simulink model "CLSfixed"  (R2023b)
settings: Solver=ode1  StartTime=0.0  StopTime=8000  FixedStep=0.5  RelTol=1e-3
libraries: Libs x311
(part 2 of 2)

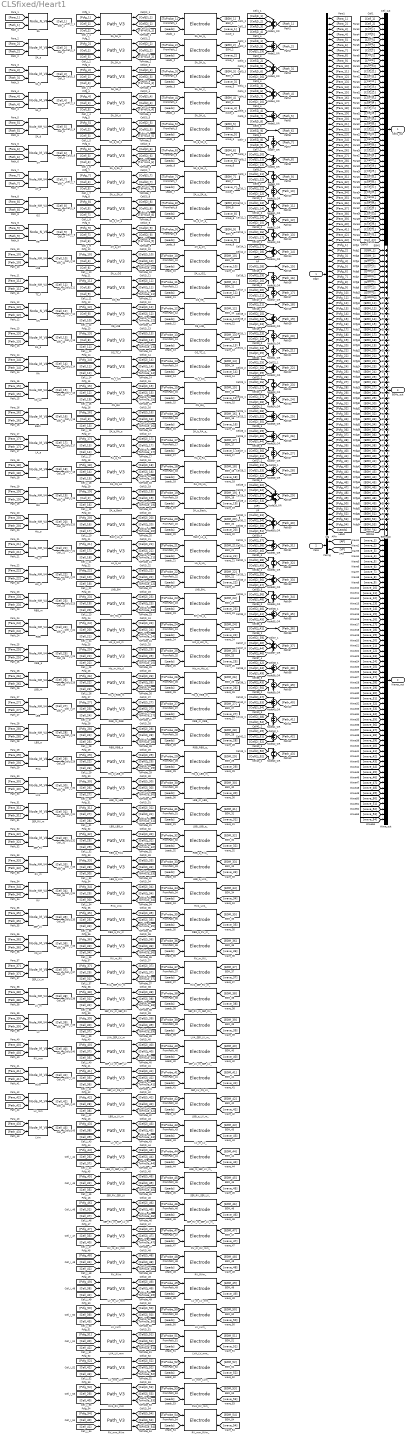
== system CLSfixed/Heart1 ==
  Cfgin : Inport
  Pace : Inport  Port=2
  BH : Libs/Node_NM_V4
  BH_His_p : Libs/Path_V3
  BH_His_p_ : Libs/Electrode
  Bach : Libs/Node_M_V4
  Bach_LA_a : Libs/Path_V3
  Bach_LA_a_ : Libs/Electrode
  CN : Libs/Node_N_V6
  CN_BH : Libs/Path_V3
  CN_BH_ : Libs/Electrode
  CS_LA : Libs/Node_NM_V4
  CS_LV : Libs/Node_M_V4
  CT : Libs/Node_M_V4
  CT_a : Libs/Node_NM_V4
  CT_a_CT : Libs/Path_V3
  CT_a_CT_ : Libs/Electrode
  Cell_out : Mux  Inputs=43
  Cfg : Demux  Outputs=[23,25,25,25,50,25,50,50,23,50,50,23,25,25,50,25,25,25,50,50,50,50,50,50,50,50,50,50,25,25,25,25,50,50,25,25,25,50,50,25,25,25,25,11,11,11,11,11,11,11,11,11,11,11,11,11,11,11,11,11,11,11,11,11,11,11,11,11,11,11,11,11,11,11,11,11,11,11,11,11,11,11,11,11,11,11,11,11,11,11,11,11,11,11,11,11,11,28]
  EGM_out : Sum  Inputs=54
  His_d : Libs/Node_NM_V4
  His_d_LBB_m : Libs/Path_V3
  His_d_LBB_m_ : Libs/Electrode
  His_d_RBB_m : Libs/Path_V3
  His_d_RBB_m_ : Libs/Electrode
  His_m : Libs/Node_NM_V4
  His_m_His_d : Libs/Path_V3
  His_m_His_d_ : Libs/Electrode
  His_p : Libs/Node_NM_V4
  His_p_His_m : Libs/Path_V3
  His_p_His_m_ : Libs/Electrode
  LA : Libs/Node_M_V4
  LA_a : Libs/Node_M_V4
  LA_a_LA : Libs/Path_V3
  LA_a_LA_ : Libs/Electrode
  LBB : Libs/Node_NM_V4
  LBB_LBB_a : Libs/Path_V3
  LBB_LBB_a_ : Libs/Electrode
  LBB_a : Libs/Node_NM_V4
  LBB_a_LVA : Libs/Path_V3
  LBB_a_LVA_ : Libs/Electrode
  LBB_a_LV_m : Libs/Path_V3
  LBB_a_LV_m_ : Libs/Electrode
  LBB_m : Libs/Node_NM_V4
  LBB_m_LBB : Libs/Path_V3
  LBB_m_LBB_ : Libs/Electrode
  LBB_m_SEP_LV_m : Libs/Path_V3
  LBB_m_SEP_LV_m_ : Libs/Electrode
  LNB : Libs/Node_NM_V4
  LNB_BH : Libs/Path_V3
  LNB_BH_ : Libs/Electrode
  LV : Libs/Node_NM_V4
  LVA : Libs/Node_M_V4
  LVA_LV_mm : Libs/Path_V3
  LVA_LV_mm_ : Libs/Electrode
  LVA_SEP_LV_m : Libs/Path_V3
  LVA_SEP_LV_m_ : Libs/Electrode
  LV_LVm : Libs/Path_V3
  LV_LVm_ : Libs/Electrode
  LV_m : Libs/Node_NM_V4
  LV_m_LV : Libs/Path_V3
  LV_m_LV_ : Libs/Electrode
  LV_m_LV_mm : Libs/Path_V3
  LV_m_LV_mm_ : Libs/Electrode
  LV_mm : Libs/Node_M_V4
  LV_mm_LVm : Libs/Path_V3
  LV_mm_LVm_ : Libs/Electrode
  LVm : Libs/Node_M_V4
  Node10_OR : Sum  Inputs=2
  Node11_OR : Sum  Inputs=2
  Node12_OR : Sum  Inputs=2
  Node13_OR : Sum  Inputs=2
  Node14_OR : Sum  Inputs=3
  Node16_OR : Sum  Inputs=2
  Node17_OR : Sum  Inputs=2
  Node19_OR : Sum  Inputs=3
  Node1_OR : Sum  Inputs=4
  Node20_OR : Sum  Inputs=2
  Node21_OR : Sum  Inputs=2
  Node22_OR : Sum  Inputs=3
  Node23_OR : Sum  Inputs=2
  Node24_OR : Sum  Inputs=2
  Node25_OR : Sum  Inputs=3
  Node26_OR : Sum  Inputs=3
  Node27_OR : Sum  Inputs=2
  Node28_OR : Sum  Inputs=3
  Node29_OR : Sum  Inputs=5
  Node2_OR : Sum  Inputs=3
  Node30_OR : Sum  Inputs=4
  Node31_OR : Sum  Inputs=3
  Node32_OR : Sum  Inputs=2
  Node33_OR : Sum  Inputs=3
  Node34_OR : Sum  Inputs=2
  Node35_OR : Sum  Inputs=3
  Node37_OR : Sum  Inputs=4
  Node38_OR : Sum  Inputs=3
  Node39_OR : Sum  Inputs=2
  Node3_OR : Sum  Inputs=4
  Node40_OR : Sum  Inputs=3
  Node41_OR : Sum  Inputs=2
  Node42_OR : Sum  Inputs=3
  Node43_OR : Sum  Inputs=2
  Node4_OR : Sum  Inputs=4
  Node5_OR : Sum  Inputs=3
  Node7_OR : Sum  Inputs=2
  Node8_OR : Sum  Inputs=3
  Node9_OR : Sum  Inputs=2
  OS : Libs/Node_NM_V4
  OS_RE : Libs/Path_V3
  OS_RE_ : Libs/Electrode
  OS_TC_f : Libs/Path_V3
  OS_TC_f_ : Libs/Electrode
  Pacing : Demux  Outputs=2
  RA : Libs/Node_M_V4
  RA_CS_LA : Libs/Path_V3
  RA_CS_LA_ : Libs/Electrode
  RA_a : Libs/Node_M_V4
  RA_a_RA : Libs/Path_V3
  RA_a_RA_ : Libs/Electrode
  RBB : Libs/Node_NM_V4
  RBB_RBB_a : Libs/Path_V3
  RBB_RBB_a_ : Libs/Electrode
  RBB_a : Libs/Node_NM_V4
  RBB_a_RVA : Libs/Path_V3
  RBB_a_RVA_ : Libs/Electrode
  RBB_a_RV_m : Libs/Path_V3
  RBB_a_RV_m_ : Libs/Electrode
  RBB_m : Libs/Node_NM_V4
  RBB_m_RBB : Libs/Path_V3
  RBB_m_RBB_ : Libs/Electrode
  RE : Libs/Node_N_V6
  RE_LNB : Libs/Path_V3
  RE_LNB_ : Libs/Electrode
  RV : Libs/Node_NM_V4
  RVA : Libs/Node_M_V4
  RVA_LVA : Libs/Path_V3
  RVA_LVA_ : Libs/Electrode
  RVA_RV_mm : Libs/Path_V3
  RVA_RV_mm_ : Libs/Electrode
  RVA_SEP_RV_m : Libs/Path_V3
  RVA_SEP_RV_m_ : Libs/Electrode
  RV_RVm : Libs/Path_V3
  RV_RVm_ : Libs/Electrode
  RV_m : Libs/Node_NM_V4
  RV_m_RV : Libs/Path_V3
  RV_m_RV_ : Libs/Electrode
  RV_m_RV_mm : Libs/Path_V3
  RV_m_RV_mm_ : Libs/Electrode
  RV_mm : Libs/Node_M_V4
  RV_mm_RVm : Libs/Path_V3
  RV_mm_RVm_ : Libs/Electrode
  RVm : Libs/Node_M_V4
  SA : Libs/Node_N_V6
  SA_SA_a : Libs/Path_V3
  SA_SA_a_ : Libs/Electrode
  SA_SA_b : Libs/Path_V3
  SA_SA_b_ : Libs/Electrode
  SA_SA_c : Libs/Path_V3
  SA_SA_c_ : Libs/Electrode
  SA_SA_d : Libs/Path_V3
  SA_SA_d_ : Libs/Electrode
  SA_a : Libs/Node_M_V4
  SA_a_Bach : Libs/Path_V3
  SA_a_Bach_ : Libs/Electrode
  SA_a_SA_b : Libs/Path_V3
  SA_a_SA_b_ : Libs/Electrode
  SA_b : Libs/Node_M_V4
  SA_b_RA_a : Libs/Path_V3
  SA_b_RA_a_ : Libs/Electrode
  SA_b_SA_c : Libs/Path_V3
  SA_b_SA_c_ : Libs/Electrode
  SA_c : Libs/Node_M_V4
  SA_c_OS : Libs/Path_V3
  SA_c_OS_ : Libs/Electrode
  SA_c_SA_d : Libs/Path_V3
  SA_c_SA_d_ : Libs/Electrode
  SA_d : Libs/Node_NM_V4
  SA_d_CT_a : Libs/Path_V3
  SA_d_CT_a_ : Libs/Electrode
  SEP_LV : Libs/Node_M_V4
  SEP_LV_CS_LV : Libs/Path_V3
  SEP_LV_CS_LV_ : Libs/Electrode
  SEP_LV_m : Libs/Node_M_V4
  SEP_LV_m_SEP_LV : Libs/Path_V3
  SEP_LV_m_SEP_LV_ : Libs/Electrode
  SEP_RV : Libs/Node_M_V4
  SEP_RV_SEP_LV : Libs/Path_V3
  SEP_RV_SEP_LV_ : Libs/Electrode
  SEP_RV_m : Libs/Node_M_V4
  SEP_RV_m_SEP_LV_m : Libs/Path_V3
  SEP_RV_m_SEP_LV_m_ : Libs/Electrode
  SEP_RV_m_SEP_RV : Libs/Path_V3
  SEP_RV_m_SEP_RV_ : Libs/Electrode
  TC_f : Libs/Node_NM_V4
  TC_f_CN : Libs/Path_V3
  TC_f_CN_ : Libs/Electrode
  Wave_out : Mux  Inputs=54
  Cells_out : Outport
  Waves_out : Outport  Port=2
  EGMs_out : Outport  Port=3
  wires:
  SA/1 -> [Cell_1]
  [Para_1] -> SA/1
  [Path_1] -> SA/2
  SA_a/1 -> [Cell_2]
  [Para_2] -> SA_a/1
  [Path_2] -> SA_a/2
  SA_b/1 -> [Cell_3]
  [Para_3] -> SA_b/1
  [Path_3] -> SA_b/2
  SA_c/1 -> [Cell_4]
  [Para_4] -> SA_c/1
  [Path_4] -> SA_c/2
  SA_d/1 -> [Cell_5]
  [Para_5] -> SA_d/1
  [Path_5] -> SA_d/2
  CT/1 -> [Cell_6]
  [Para_6] -> CT/1
  [Path_6] -> CT/2
  CT_a/1 -> [Cell_7]
  [Para_7] -> CT_a/1
  [Path_7] -> CT_a/2
  OS/1 -> [Cell_8]
  [Para_8] -> OS/1
  [Path_8] -> OS/2
  RE/1 -> [Cell_9]
  [Para_9] -> RE/1
  [Path_9] -> RE/2
  LNB/1 -> [Cell_10]
  [Para_10] -> LNB/1
  [Path_10] -> LNB/2
  TC_f/1 -> [Cell_11]
  [Para_11] -> TC_f/1
  [Path_11] -> TC_f/2
  CN/1 -> [Cell_12]
  [Para_12] -> CN/1
  [Path_12] -> CN/2
  RA_a/1 -> [Cell_13]
  [Para_13] -> RA_a/1
  [Path_13] -> RA_a/2
  RA/1 -> [Cell_14]
  [Para_14] -> RA/1
  [Path_14] -> RA/2
  CS_LA/1 -> [Cell_15]
  [Para_15] -> CS_LA/1
  [Path_15] -> CS_LA/2
  Bach/1 -> [Cell_16]
  [Para_16] -> Bach/1
  [Path_16] -> Bach/2
  LA_a/1 -> [Cell_17]
  [Para_17] -> LA_a/1
  [Path_17] -> LA_a/2
  LA/1 -> [Cell_18]
  [Para_18] -> LA/1
  [Path_18] -> LA/2
  BH/1 -> [Cell_19]
  [Para_19] -> BH/1
  [Path_19] -> BH/2
  His_p/1 -> [Cell_20]
  [Para_20] -> His_p/1
  [Path_20] -> His_p/2
  His_m/1 -> [Cell_21]
  [Para_21] -> His_m/1
  [Path_21] -> His_m/2
  His_d/1 -> [Cell_22]
  [Para_22] -> His_d/1
  [Path_22] -> His_d/2
  RBB_m/1 -> [Cell_23]
  [Para_23] -> RBB_m/1
  [Path_23] -> RBB_m/2
  RBB/1 -> [Cell_24]
  [Para_24] -> RBB/1
  [Path_24] -> RBB/2
  RBB_a/1 -> [Cell_25]
  [Para_25] -> RBB_a/1
  [Path_25] -> RBB_a/2
  LBB_m/1 -> [Cell_26]
  [Para_26] -> LBB_m/1
  [Path_26] -> LBB_m/2
  LBB/1 -> [Cell_27]
  [Para_27] -> LBB/1
  [Path_27] -> LBB/2
  LBB_a/1 -> [Cell_28]
  [Para_28] -> LBB_a/1
  [Path_28] -> LBB_a/2
  RVA/1 -> [Cell_29]
  [Para_29] -> RVA/1
  [Path_29] -> RVA/2
  LVA/1 -> [Cell_30]
  [Para_30] -> LVA/1
  [Path_30] -> LVA/2
  SEP_RV_m/1 -> [Cell_31]
  [Para_31] -> SEP_RV_m/1
  [Path_31] -> SEP_RV_m/2
  SEP_RV/1 -> [Cell_32]
  [Para_32] -> SEP_RV/1
  [Path_32] -> SEP_RV/2
  RV_m/1 -> [Cell_33]
  [Para_33] -> RV_m/1
  [Path_33] -> RV_m/2
  RV/1 -> [Cell_34]
  [Para_34] -> RV/1
  [Path_34] -> RV/2
  SEP_LV/1 -> [Cell_35]
  [Para_35] -> SEP_LV/1
  [Path_35] -> SEP_LV/2
  CS_LV/1 -> [Cell_36]
  [Para_36] -> CS_LV/1
  [Path_36] -> CS_LV/2
  SEP_LV_m/1 -> [Cell_37]
  [Para_37] -> SEP_LV_m/1
  [Path_37] -> SEP_LV_m/2
  LV_m/1 -> [Cell_38]
  [Para_38] -> LV_m/1
  [Path_38] -> LV_m/2
  LV/1 -> [Cell_39]
  [Para_39] -> LV/1
  [Path_39] -> LV/2
  RV_mm/1 -> [Cell_40]
  [Para_40] -> RV_mm/1
  [Path_40] -> RV_mm/2
  RVm/1 -> [Cell_41]
  [Para_41] -> RVm/1
  [Path_41] -> RVm/2
  LV_mm/1 -> [Cell_42]
  [Para_42] -> LV_mm/1
  [Path_42] -> LV_mm/2
  LVm/1 -> [Cell_43]
  [Para_43] -> LVm/1
  [Path_43] -> LVm/2
  SA_SA_a/1 -> [Cellj2i_1]
  SA_SA_a/2 -> [Celli2j_1]
  SA_SA_a/3 -> [ToProbe_1]
  [Pcfg_1] -> SA_SA_a/1
  [Cell_1] -> SA_SA_a/2
  [Cell_2] -> SA_SA_a/3
  SA_SA_b/1 -> [Cellj2i_2]
  SA_SA_b/2 -> [Celli2j_2]
  SA_SA_b/3 -> [ToProbe_2]
  [Pcfg_2] -> SA_SA_b/1
  [Cell_1] -> SA_SA_b/2
  [Cell_3] -> SA_SA_b/3
  SA_SA_c/1 -> [Cellj2i_3]
  SA_SA_c/2 -> [Celli2j_3]
  SA_SA_c/3 -> [ToProbe_3]
  [Pcfg_3] -> SA_SA_c/1
  [Cell_1] -> SA_SA_c/2
  [Cell_4] -> SA_SA_c/3
  SA_SA_d/1 -> [Cellj2i_4]
  SA_SA_d/2 -> [Celli2j_4]
  SA_SA_d/3 -> [ToProbe_4]
  [Pcfg_4] -> SA_SA_d/1
  [Cell_1] -> SA_SA_d/2
  [Cell_5] -> SA_SA_d/3
  SA_a_SA_b/1 -> [Cellj2i_5]
  SA_a_SA_b/2 -> [Celli2j_5]
  SA_a_SA_b/3 -> [ToProbe_5]
  [Pcfg_5] -> SA_a_SA_b/1
  [Cell_2] -> SA_a_SA_b/2
  [Cell_3] -> SA_a_SA_b/3
  SA_b_SA_c/1 -> [Cellj2i_6]
  SA_b_SA_c/2 -> [Celli2j_6]
  SA_b_SA_c/3 -> [ToProbe_6]
  [Pcfg_6] -> SA_b_SA_c/1
  [Cell_3] -> SA_b_SA_c/2
  [Cell_4] -> SA_b_SA_c/3
  SA_c_SA_d/1 -> [Cellj2i_7]
  SA_c_SA_d/2 -> [Celli2j_7]
  SA_c_SA_d/3 -> [ToProbe_7]
  [Pcfg_7] -> SA_c_SA_d/1
  [Cell_4] -> SA_c_SA_d/2
  [Cell_5] -> SA_c_SA_d/3
  SA_d_CT_a/1 -> [Cellj2i_8]
  SA_d_CT_a/2 -> [Celli2j_8]
  SA_d_CT_a/3 -> [ToProbe_8]
  [Pcfg_8] -> SA_d_CT_a/1
  [Cell_5] -> SA_d_CT_a/2
  [Cell_7] -> SA_d_CT_a/3
  CT_a_CT/1 -> [Cellj2i_9]
  CT_a_CT/2 -> [Celli2j_9]
  CT_a_CT/3 -> [ToProbe_9]
  [Pcfg_9] -> CT_a_CT/1
  [Cell_7] -> CT_a_CT/2
  [Cell_6] -> CT_a_CT/3
  SA_c_OS/1 -> [Cellj2i_10]
  SA_c_OS/2 -> [Celli2j_10]
  SA_c_OS/3 -> [ToProbe_10]
  [Pcfg_10] -> SA_c_OS/1
  [Cell_4] -> SA_c_OS/2
  [Cell_8] -> SA_c_OS/3
  OS_RE/1 -> [Cellj2i_11]
  OS_RE/2 -> [Celli2j_11]
  OS_RE/3 -> [ToProbe_11]
  [Pcfg_11] -> OS_RE/1
  [Cell_8] -> OS_RE/2
  [Cell_9] -> OS_RE/3
  RE_LNB/1 -> [Cellj2i_12]
  RE_LNB/2 -> [Celli2j_12]
  RE_LNB/3 -> [ToProbe_12]
  [Pcfg_12] -> RE_LNB/1
  [Cell_9] -> RE_LNB/2
  [Cell_10] -> RE_LNB/3
  OS_TC_f/1 -> [Cellj2i_13]
  OS_TC_f/2 -> [Celli2j_13]
  OS_TC_f/3 -> [ToProbe_13]
  [Pcfg_13] -> OS_TC_f/1
  [Cell_8] -> OS_TC_f/2
  [Cell_11] -> OS_TC_f/3
  TC_f_CN/1 -> [Cellj2i_14]
  TC_f_CN/2 -> [Celli2j_14]
  TC_f_CN/3 -> [ToProbe_14]
  [Pcfg_14] -> TC_f_CN/1
  [Cell_11] -> TC_f_CN/2
  [Cell_12] -> TC_f_CN/3
  CN_BH/1 -> [Cellj2i_15]
  CN_BH/2 -> [Celli2j_15]
  CN_BH/3 -> [ToProbe_15]
  [Pcfg_15] -> CN_BH/1
  [Cell_12] -> CN_BH/2
  [Cell_19] -> CN_BH/3
  SA_b_RA_a/1 -> [Cellj2i_16]
  SA_b_RA_a/2 -> [Celli2j_16]
  SA_b_RA_a/3 -> [ToProbe_16]
  [Pcfg_16] -> SA_b_RA_a/1
  [Cell_3] -> SA_b_RA_a/2
  [Cell_13] -> SA_b_RA_a/3
  RA_a_RA/1 -> [Cellj2i_17]
  RA_a_RA/2 -> [Celli2j_17]
  RA_a_RA/3 -> [ToProbe_17]
  [Pcfg_17] -> RA_a_RA/1
  [Cell_13] -> RA_a_RA/2
  [Cell_14] -> RA_a_RA/3
  RA_CS_LA/1 -> [Cellj2i_18]
  RA_CS_LA/2 -> [Celli2j_18]
  RA_CS_LA/3 -> [ToProbe_18]
  [Pcfg_18] -> RA_CS_LA/1
  [Cell_14] -> RA_CS_LA/2
  [Cell_15] -> RA_CS_LA/3
  SA_a_Bach/1 -> [Cellj2i_19]
  SA_a_Bach/2 -> [Celli2j_19]
  SA_a_Bach/3 -> [ToProbe_19]
  [Pcfg_19] -> SA_a_Bach/1
  [Cell_2] -> SA_a_Bach/2
  [Cell_16] -> SA_a_Bach/3
  Bach_LA_a/1 -> [Cellj2i_20]
  Bach_LA_a/2 -> [Celli2j_20]
  Bach_LA_a/3 -> [ToProbe_20]
  [Pcfg_20] -> Bach_LA_a/1
  [Cell_16] -> Bach_LA_a/2
  [Cell_17] -> Bach_LA_a/3
  LA_a_LA/1 -> [Cellj2i_21]
  LA_a_LA/2 -> [Celli2j_21]
  LA_a_LA/3 -> [ToProbe_21]
  [Pcfg_21] -> LA_a_LA/1
  [Cell_17] -> LA_a_LA/2
  [Cell_18] -> LA_a_LA/3
  LNB_BH/1 -> [Cellj2i_22]
  LNB_BH/2 -> [Celli2j_22]
  LNB_BH/3 -> [ToProbe_22]
  [Pcfg_22] -> LNB_BH/1
  [Cell_10] -> LNB_BH/2
  [Cell_19] -> LNB_BH/3
  BH_His_p/1 -> [Cellj2i_23]
  BH_His_p/2 -> [Celli2j_23]
  BH_His_p/3 -> [ToProbe_23]
  [Pcfg_23] -> BH_His_p/1
  [Cell_19] -> BH_His_p/2
  [Cell_20] -> BH_His_p/3
  His_p_His_m/1 -> [Cellj2i_24]
  His_p_His_m/2 -> [Celli2j_24]
  His_p_His_m/3 -> [ToProbe_24]
  [Pcfg_24] -> His_p_His_m/1
  [Cell_20] -> His_p_His_m/2
  [Cell_21] -> His_p_His_m/3
  His_m_His_d/1 -> [Cellj2i_25]
  His_m_His_d/2 -> [Celli2j_25]
  His_m_His_d/3 -> [ToProbe_25]
  [Pcfg_25] -> His_m_His_d/1
  [Cell_21] -> His_m_His_d/2
  [Cell_22] -> His_m_His_d/3
  His_d_RBB_m/1 -> [Cellj2i_26]
  His_d_RBB_m/2 -> [Celli2j_26]
  His_d_RBB_m/3 -> [ToProbe_26]
  [Pcfg_26] -> His_d_RBB_m/1
  [Cell_22] -> His_d_RBB_m/2
  [Cell_23] -> His_d_RBB_m/3
  RBB_m_RBB/1 -> [Cellj2i_27]
  RBB_m_RBB/2 -> [Celli2j_27]
  RBB_m_RBB/3 -> [ToProbe_27]
  [Pcfg_27] -> RBB_m_RBB/1
  [Cell_23] -> RBB_m_RBB/2
  [Cell_24] -> RBB_m_RBB/3
  RBB_RBB_a/1 -> [Cellj2i_28]
  RBB_RBB_a/2 -> [Celli2j_28]
  RBB_RBB_a/3 -> [ToProbe_28]
  [Pcfg_28] -> RBB_RBB_a/1
  [Cell_24] -> RBB_RBB_a/2
  [Cell_25] -> RBB_RBB_a/3
  His_d_LBB_m/1 -> [Cellj2i_29]
  His_d_LBB_m/2 -> [Celli2j_29]
  His_d_LBB_m/3 -> [ToProbe_29]
  [Pcfg_29] -> His_d_LBB_m/1
  [Cell_22] -> His_d_LBB_m/2
  [Cell_26] -> His_d_LBB_m/3
  LBB_m_LBB/1 -> [Cellj2i_30]
  LBB_m_LBB/2 -> [Celli2j_30]
  LBB_m_LBB/3 -> [ToProbe_30]
  [Pcfg_30] -> LBB_m_LBB/1
  [Cell_26] -> LBB_m_LBB/2
  [Cell_27] -> LBB_m_LBB/3
  LBB_LBB_a/1 -> [Cellj2i_31]
  LBB_LBB_a/2 -> [Celli2j_31]
  LBB_LBB_a/3 -> [ToProbe_31]
  [Pcfg_31] -> LBB_LBB_a/1
  [Cell_27] -> LBB_LBB_a/2
  [Cell_28] -> LBB_LBB_a/3
  RBB_a_RVA/1 -> [Cellj2i_32]
  RBB_a_RVA/2 -> [Celli2j_32]
  RBB_a_RVA/3 -> [ToProbe_32]
  [Pcfg_32] -> RBB_a_RVA/1
  [Cell_25] -> RBB_a_RVA/2
  [Cell_29] -> RBB_a_RVA/3
  LBB_a_LVA/1 -> [Cellj2i_33]
  LBB_a_LVA/2 -> [Celli2j_33]
  LBB_a_LVA/3 -> [ToProbe_33]
  [Pcfg_33] -> LBB_a_LVA/1
  [Cell_28] -> LBB_a_LVA/2
  [Cell_30] -> LBB_a_LVA/3
  RVA_LVA/1 -> [Cellj2i_34]
  RVA_LVA/2 -> [Celli2j_34]
  RVA_LVA/3 -> [ToProbe_34]
  [Pcfg_34] -> RVA_LVA/1
  [Cell_29] -> RVA_LVA/2
  [Cell_30] -> RVA_LVA/3
  RBB_a_RV_m/1 -> [Cellj2i_35]
  RBB_a_RV_m/2 -> [Celli2j_35]
  RBB_a_RV_m/3 -> [ToProbe_35]
  [Pcfg_35] -> RBB_a_RV_m/1
  [Cell_25] -> RBB_a_RV_m/2
  [Cell_33] -> RBB_a_RV_m/3
  RV_m_RV/1 -> [Cellj2i_36]
  RV_m_RV/2 -> [Celli2j_36]
  RV_m_RV/3 -> [ToProbe_36]
  [Pcfg_36] -> RV_m_RV/1
  [Cell_33] -> RV_m_RV/2
  [Cell_34] -> RV_m_RV/3
  RVA_SEP_RV_m/1 -> [Cellj2i_37]
  RVA_SEP_RV_m/2 -> [Celli2j_37]
  RVA_SEP_RV_m/3 -> [ToProbe_37]
  [Pcfg_37] -> RVA_SEP_RV_m/1
  [Cell_29] -> RVA_SEP_RV_m/2
  [Cell_31] -> RVA_SEP_RV_m/3
  SEP_RV_m_SEP_RV/1 -> [Cellj2i_38]
  SEP_RV_m_SEP_RV/2 -> [Celli2j_38]
  SEP_RV_m_SEP_RV/3 -> [ToProbe_38]
  [Pcfg_38] -> SEP_RV_m_SEP_RV/1
  [Cell_31] -> SEP_RV_m_SEP_RV/2
  [Cell_32] -> SEP_RV_m_SEP_RV/3
  LVA_SEP_LV_m/1 -> [Cellj2i_39]
  LVA_SEP_LV_m/2 -> [Celli2j_39]
  LVA_SEP_LV_m/3 -> [ToProbe_39]
  [Pcfg_39] -> LVA_SEP_LV_m/1
  [Cell_30] -> LVA_SEP_LV_m/2
  [Cell_37] -> LVA_SEP_LV_m/3
  SEP_LV_m_SEP_LV/1 -> [Cellj2i_40]
  SEP_LV_m_SEP_LV/2 -> [Celli2j_40]
  SEP_LV_m_SEP_LV/3 -> [ToProbe_40]
  [Pcfg_40] -> SEP_LV_m_SEP_LV/1
  [Cell_37] -> SEP_LV_m_SEP_LV/2
  [Cell_35] -> SEP_LV_m_SEP_LV/3
  SEP_LV_CS_LV/1 -> [Cellj2i_41]
  SEP_LV_CS_LV/2 -> [Celli2j_41]
  SEP_LV_CS_LV/3 -> [ToProbe_41]
  [Pcfg_41] -> SEP_LV_CS_LV/1
  [Cell_35] -> SEP_LV_CS_LV/2
  [Cell_36] -> SEP_LV_CS_LV/3
  LBB_a_LV_m/1 -> [Cellj2i_42]
  LBB_a_LV_m/2 -> [Celli2j_42]
  LBB_a_LV_m/3 -> [ToProbe_42]
  [Pcfg_42] -> LBB_a_LV_m/1
  [Cell_28] -> LBB_a_LV_m/2
  [Cell_38] -> LBB_a_LV_m/3
  LV_m_LV/1 -> [Cellj2i_43]
  LV_m_LV/2 -> [Celli2j_43]
  LV_m_LV/3 -> [ToProbe_43]
  [Pcfg_43] -> LV_m_LV/1
  [Cell_38] -> LV_m_LV/2
  [Cell_39] -> LV_m_LV/3
  LBB_m_SEP_LV_m/1 -> [Cellj2i_44]
  LBB_m_SEP_LV_m/2 -> [Celli2j_44]
  LBB_m_SEP_LV_m/3 -> [ToProbe_44]
  [Pcfg_44] -> LBB_m_SEP_LV_m/1
  [Cell_26] -> LBB_m_SEP_LV_m/2
  [Cell_37] -> LBB_m_SEP_LV_m/3
  SEP_RV_SEP_LV/1 -> [Cellj2i_45]
  SEP_RV_SEP_LV/2 -> [Celli2j_45]
  SEP_RV_SEP_LV/3 -> [ToProbe_45]
  [Pcfg_45] -> SEP_RV_SEP_LV/1
  [Cell_32] -> SEP_RV_SEP_LV/2
  [Cell_35] -> SEP_RV_SEP_LV/3
  SEP_RV_m_SEP_LV_m/1 -> [Cellj2i_46]
  SEP_RV_m_SEP_LV_m/2 -> [Celli2j_46]
  SEP_RV_m_SEP_LV_m/3 -> [ToProbe_46]
  [Pcfg_46] -> SEP_RV_m_SEP_LV_m/1
  [Cell_31] -> SEP_RV_m_SEP_LV_m/2
  [Cell_37] -> SEP_RV_m_SEP_LV_m/3
  RV_m_RV_mm/1 -> [Cellj2i_47]
  RV_m_RV_mm/2 -> [Celli2j_47]
  RV_m_RV_mm/3 -> [ToProbe_47]
  [Pcfg_47] -> RV_m_RV_mm/1
  [Cell_33] -> RV_m_RV_mm/2
  [Cell_40] -> RV_m_RV_mm/3
  RV_RVm/1 -> [Cellj2i_48]
  RV_RVm/2 -> [Celli2j_48]
  RV_RVm/3 -> [ToProbe_48]
  [Pcfg_48] -> RV_RVm/1
  [Cell_34] -> RV_RVm/2
  [Cell_41] -> RV_RVm/3
  LV_m_LV_mm/1 -> [Cellj2i_49]
  LV_m_LV_mm/2 -> [Celli2j_49]
  LV_m_LV_mm/3 -> [ToProbe_49]
  [Pcfg_49] -> LV_m_LV_mm/1
  [Cell_38] -> LV_m_LV_mm/2
  [Cell_42] -> LV_m_LV_mm/3
  LV_LVm/1 -> [Cellj2i_50]
  LV_LVm/2 -> [Celli2j_50]
  LV_LVm/3 -> [ToProbe_50]
  [Pcfg_50] -> LV_LVm/1
  [Cell_39] -> LV_LVm/2
  [Cell_43] -> LV_LVm/3
  LVA_LV_mm/1 -> [Cellj2i_51]
  LVA_LV_mm/2 -> [Celli2j_51]
  LVA_LV_mm/3 -> [ToProbe_51]
  [Pcfg_51] -> LVA_LV_mm/1
  [Cell_30] -> LVA_LV_mm/2
  [Cell_42] -> LVA_LV_mm/3
  LV_mm_LVm/1 -> [Cellj2i_52]
  LV_mm_LVm/2 -> [Celli2j_52]
  LV_mm_LVm/3 -> [ToProbe_52]
  [Pcfg_52] -> LV_mm_LVm/1
  [Cell_42] -> LV_mm_LVm/2
  [Cell_43] -> LV_mm_LVm/3
  RVA_RV_mm/1 -> [Cellj2i_53]
  RVA_RV_mm/2 -> [Celli2j_53]
  RVA_RV_mm/3 -> [ToProbe_53]
  [Pcfg_53] -> RVA_RV_mm/1
  [Cell_29] -> RVA_RV_mm/2
  [Cell_40] -> RVA_RV_mm/3
  RV_mm_RVm/1 -> [Cellj2i_54]
  RV_mm_RVm/2 -> [Celli2j_54]
  RV_mm_RVm/3 -> [ToProbe_54]
  [Pcfg_54] -> RV_mm_RVm/1
  [Cell_40] -> RV_mm_RVm/2
  [Cell_41] -> RV_mm_RVm/3
  SA_SA_a_/1 -> [EGM_1]
  SA_SA_a_/2 -> [wave_1]
  [ToProbe_1] -> SA_SA_a_/1
  [Leads] -> SA_SA_a_/2
  SA_SA_b_/1 -> [EGM_2]
  SA_SA_b_/2 -> [wave_2]
  [ToProbe_2] -> SA_SA_b_/1
  [Leads] -> SA_SA_b_/2
  SA_SA_c_/1 -> [EGM_3]
  SA_SA_c_/2 -> [wave_3]
  [ToProbe_3] -> SA_SA_c_/1
  [Leads] -> SA_SA_c_/2
  SA_SA_d_/1 -> [EGM_4]
  SA_SA_d_/2 -> [wave_4]
  [ToProbe_4] -> SA_SA_d_/1
  [Leads] -> SA_SA_d_/2
  SA_a_SA_b_/1 -> [EGM_5]
  SA_a_SA_b_/2 -> [wave_5]
  [ToProbe_5] -> SA_a_SA_b_/1
  [Leads] -> SA_a_SA_b_/2
  SA_b_SA_c_/1 -> [EGM_6]
  SA_b_SA_c_/2 -> [wave_6]
  [ToProbe_6] -> SA_b_SA_c_/1
  [Leads] -> SA_b_SA_c_/2
  SA_c_SA_d_/1 -> [EGM_7]
  SA_c_SA_d_/2 -> [wave_7]
  [ToProbe_7] -> SA_c_SA_d_/1
  [Leads] -> SA_c_SA_d_/2
  SA_d_CT_a_/1 -> [EGM_8]
  SA_d_CT_a_/2 -> [wave_8]
  [ToProbe_8] -> SA_d_CT_a_/1
  [Leads] -> SA_d_CT_a_/2
  CT_a_CT_/1 -> [EGM_9]
  CT_a_CT_/2 -> [wave_9]
  [ToProbe_9] -> CT_a_CT_/1
  [Leads] -> CT_a_CT_/2
  SA_c_OS_/1 -> [EGM_10]
  SA_c_OS_/2 -> [wave_10]
  [ToProbe_10] -> SA_c_OS_/1
  [Leads] -> SA_c_OS_/2
  OS_RE_/1 -> [EGM_11]
  OS_RE_/2 -> [wave_11]
  [ToProbe_11] -> OS_RE_/1
  [Leads] -> OS_RE_/2
  RE_LNB_/1 -> [EGM_12]
  RE_LNB_/2 -> [wave_12]
  [ToProbe_12] -> RE_LNB_/1
  [Leads] -> RE_LNB_/2
  OS_TC_f_/1 -> [EGM_13]
  OS_TC_f_/2 -> [wave_13]
  [ToProbe_13] -> OS_TC_f_/1
  [Leads] -> OS_TC_f_/2
  TC_f_CN_/1 -> [EGM_14]
  TC_f_CN_/2 -> [wave_14]
  [ToProbe_14] -> TC_f_CN_/1
  [Leads] -> TC_f_CN_/2
  CN_BH_/1 -> [EGM_15]
  CN_BH_/2 -> [wave_15]
  [ToProbe_15] -> CN_BH_/1
  [Leads] -> CN_BH_/2
  SA_b_RA_a_/1 -> [EGM_16]
  SA_b_RA_a_/2 -> [wave_16]
  [ToProbe_16] -> SA_b_RA_a_/1
  [Leads] -> SA_b_RA_a_/2
  RA_a_RA_/1 -> [EGM_17]
  RA_a_RA_/2 -> [wave_17]
  [ToProbe_17] -> RA_a_RA_/1
  [Leads] -> RA_a_RA_/2
  RA_CS_LA_/1 -> [EGM_18]
  RA_CS_LA_/2 -> [wave_18]
  [ToProbe_18] -> RA_CS_LA_/1
  [Leads] -> RA_CS_LA_/2
  SA_a_Bach_/1 -> [EGM_19]
  SA_a_Bach_/2 -> [wave_19]
  [ToProbe_19] -> SA_a_Bach_/1
  [Leads] -> SA_a_Bach_/2
  Bach_LA_a_/1 -> [EGM_20]
  Bach_LA_a_/2 -> [wave_20]
  [ToProbe_20] -> Bach_LA_a_/1
  [Leads] -> Bach_LA_a_/2
  LA_a_LA_/1 -> [EGM_21]
  LA_a_LA_/2 -> [wave_21]
  [ToProbe_21] -> LA_a_LA_/1
  [Leads] -> LA_a_LA_/2
  LNB_BH_/1 -> [EGM_22]
  LNB_BH_/2 -> [wave_22]
  [ToProbe_22] -> LNB_BH_/1
  [Leads] -> LNB_BH_/2
  BH_His_p_/1 -> [EGM_23]
  BH_His_p_/2 -> [wave_23]
  [ToProbe_23] -> BH_His_p_/1
  [Leads] -> BH_His_p_/2
  His_p_His_m_/1 -> [EGM_24]
  His_p_His_m_/2 -> [wave_24]
  [ToProbe_24] -> His_p_His_m_/1
  [Leads] -> His_p_His_m_/2
  His_m_His_d_/1 -> [EGM_25]
  His_m_His_d_/2 -> [wave_25]
  [ToProbe_25] -> His_m_His_d_/1
  [Leads] -> His_m_His_d_/2
  His_d_RBB_m_/1 -> [EGM_26]
  His_d_RBB_m_/2 -> [wave_26]
  [ToProbe_26] -> His_d_RBB_m_/1
  [Leads] -> His_d_RBB_m_/2
  RBB_m_RBB_/1 -> [EGM_27]
  RBB_m_RBB_/2 -> [wave_27]
  [ToProbe_27] -> RBB_m_RBB_/1
  [Leads] -> RBB_m_RBB_/2
  RBB_RBB_a_/1 -> [EGM_28]
  RBB_RBB_a_/2 -> [wave_28]
  [ToProbe_28] -> RBB_RBB_a_/1
  [Leads] -> RBB_RBB_a_/2
  His_d_LBB_m_/1 -> [EGM_29]
  His_d_LBB_m_/2 -> [wave_29]
  [ToProbe_29] -> His_d_LBB_m_/1
  [Leads] -> His_d_LBB_m_/2
  LBB_m_LBB_/1 -> [EGM_30]
  LBB_m_LBB_/2 -> [wave_30]
  [ToProbe_30] -> LBB_m_LBB_/1
  [Leads] -> LBB_m_LBB_/2
  LBB_LBB_a_/1 -> [EGM_31]
  LBB_LBB_a_/2 -> [wave_31]
  [ToProbe_31] -> LBB_LBB_a_/1
  [Leads] -> LBB_LBB_a_/2
  RBB_a_RVA_/1 -> [EGM_32]
  RBB_a_RVA_/2 -> [wave_32]
  [ToProbe_32] -> RBB_a_RVA_/1
  [Leads] -> RBB_a_RVA_/2
  LBB_a_LVA_/1 -> [EGM_33]
  LBB_a_LVA_/2 -> [wave_33]
  [ToProbe_33] -> LBB_a_LVA_/1
  [Leads] -> LBB_a_LVA_/2
  RVA_LVA_/1 -> [EGM_34]
  RVA_LVA_/2 -> [wave_34]
  [ToProbe_34] -> RVA_LVA_/1
  [Leads] -> RVA_LVA_/2
  RBB_a_RV_m_/1 -> [EGM_35]
  RBB_a_RV_m_/2 -> [wave_35]
  [ToProbe_35] -> RBB_a_RV_m_/1
  [Leads] -> RBB_a_RV_m_/2
  RV_m_RV_/1 -> [EGM_36]
  RV_m_RV_/2 -> [wave_36]
  [ToProbe_36] -> RV_m_RV_/1
  [Leads] -> RV_m_RV_/2
  RVA_SEP_RV_m_/1 -> [EGM_37]
  RVA_SEP_RV_m_/2 -> [wave_37]
  [ToProbe_37] -> RVA_SEP_RV_m_/1
  [Leads] -> RVA_SEP_RV_m_/2
  SEP_RV_m_SEP_RV_/1 -> [EGM_38]
  SEP_RV_m_SEP_RV_/2 -> [wave_38]
  [ToProbe_38] -> SEP_RV_m_SEP_RV_/1
  [Leads] -> SEP_RV_m_SEP_RV_/2
  LVA_SEP_LV_m_/1 -> [EGM_39]
  LVA_SEP_LV_m_/2 -> [wave_39]
  [ToProbe_39] -> LVA_SEP_LV_m_/1
  [Leads] -> LVA_SEP_LV_m_/2
  SEP_LV_m_SEP_LV_/1 -> [EGM_40]
  SEP_LV_m_SEP_LV_/2 -> [wave_40]
  [ToProbe_40] -> SEP_LV_m_SEP_LV_/1
  [Leads] -> SEP_LV_m_SEP_LV_/2
  SEP_LV_CS_LV_/1 -> [EGM_41]
  SEP_LV_CS_LV_/2 -> [wave_41]
  [ToProbe_41] -> SEP_LV_CS_LV_/1
  [Leads] -> SEP_LV_CS_LV_/2
  LBB_a_LV_m_/1 -> [EGM_42]
  LBB_a_LV_m_/2 -> [wave_42]
  [ToProbe_42] -> LBB_a_LV_m_/1
  [Leads] -> LBB_a_LV_m_/2
  LV_m_LV_/1 -> [EGM_43]
  LV_m_LV_/2 -> [wave_43]
  [ToProbe_43] -> LV_m_LV_/1
  [Leads] -> LV_m_LV_/2
  LBB_m_SEP_LV_m_/1 -> [EGM_44]
  LBB_m_SEP_LV_m_/2 -> [wave_44]
  [ToProbe_44] -> LBB_m_SEP_LV_m_/1
  [Leads] -> LBB_m_SEP_LV_m_/2
  SEP_RV_SEP_LV_/1 -> [EGM_45]
  SEP_RV_SEP_LV_/2 -> [wave_45]
  [ToProbe_45] -> SEP_RV_SEP_LV_/1
  [Leads] -> SEP_RV_SEP_LV_/2
  SEP_RV_m_SEP_LV_m_/1 -> [EGM_46]
  SEP_RV_m_SEP_LV_m_/2 -> [wave_46]
  [ToProbe_46] -> SEP_RV_m_SEP_LV_m_/1
  [Leads] -> SEP_RV_m_SEP_LV_m_/2
  RV_m_RV_mm_/1 -> [EGM_47]
  RV_m_RV_mm_/2 -> [wave_47]
  [ToProbe_47] -> RV_m_RV_mm_/1
  [Leads] -> RV_m_RV_mm_/2
  RV_RVm_/1 -> [EGM_48]
  RV_RVm_/2 -> [wave_48]
  [ToProbe_48] -> RV_RVm_/1
  [Leads] -> RV_RVm_/2
  LV_m_LV_mm_/1 -> [EGM_49]
  LV_m_LV_mm_/2 -> [wave_49]
  [ToProbe_49] -> LV_m_LV_mm_/1
  [Leads] -> LV_m_LV_mm_/2
  LV_LVm_/1 -> [EGM_50]
  LV_LVm_/2 -> [wave_50]
  [ToProbe_50] -> LV_LVm_/1
  [Leads] -> LV_LVm_/2
  LVA_LV_mm_/1 -> [EGM_51]
  LVA_LV_mm_/2 -> [wave_51]
  [ToProbe_51] -> LVA_LV_mm_/1
  [Leads] -> LVA_LV_mm_/2
  LV_mm_LVm_/1 -> [EGM_52]
  LV_mm_LVm_/2 -> [wave_52]
  [ToProbe_52] -> LV_mm_LVm_/1
  [Leads] -> LV_mm_LVm_/2
  RVA_RV_mm_/1 -> [EGM_53]
  RVA_RV_mm_/2 -> [wave_53]
  [ToProbe_53] -> RVA_RV_mm_/1
  [Leads] -> RVA_RV_mm_/2
  RV_mm_RVm_/1 -> [EGM_54]
  RV_mm_RVm_/2 -> [wave_54]
  [ToProbe_54] -> RV_mm_RVm_/1
  [Leads] -> RV_mm_RVm_/2
  [Cellj2i_1] -> Node1_OR/1
  [Cellj2i_2] -> Node1_OR/2
  [Cellj2i_3] -> Node1_OR/3
  [Cellj2i_4] -> Node1_OR/4
  Node1_OR/1 -> [Path_1]
  [Celli2j_1] -> Node2_OR/1
  [Cellj2i_5] -> Node2_OR/2
  [Cellj2i_19] -> Node2_OR/3
  Node2_OR/1 -> [Path_2]
  [Celli2j_2] -> Node3_OR/1
  [Celli2j_5] -> Node3_OR/2
  [Cellj2i_6] -> Node3_OR/3
  [Cellj2i_16] -> Node3_OR/4
  Node3_OR/1 -> [Path_3]
  [Celli2j_3] -> Node4_OR/1
  [Celli2j_6] -> Node4_OR/2
  [Cellj2i_7] -> Node4_OR/3
  [Cellj2i_10] -> Node4_OR/4
  Node4_OR/1 -> [Path_4]
  [Celli2j_4] -> Node5_OR/1
  [Celli2j_7] -> Node5_OR/2
  [Cellj2i_8] -> Node5_OR/3
  Node5_OR/1 -> [Path_5]
  [Celli2j_9] -> [Path_6]
  [Celli2j_8] -> Node7_OR/1
  [Cellj2i_9] -> Node7_OR/2
  Node7_OR/1 -> [Path_7]
  [Celli2j_10] -> Node8_OR/1
  [Cellj2i_11] -> Node8_OR/2
  [Cellj2i_13] -> Node8_OR/3
  Node8_OR/1 -> [Path_8]
  [Celli2j_11] -> Node9_OR/1
  [Cellj2i_12] -> Node9_OR/2
  Node9_OR/1 -> [Path_9]
  [Celli2j_12] -> Node10_OR/1
  [Cellj2i_22] -> Node10_OR/2
  Node10_OR/1 -> [Path_10]
  [Celli2j_13] -> Node11_OR/1
  [Cellj2i_14] -> Node11_OR/2
  Node11_OR/1 -> [Path_11]
  [Celli2j_14] -> Node12_OR/1
  [Cellj2i_15] -> Node12_OR/2
  Node12_OR/1 -> [Path_12]
  [Celli2j_16] -> Node13_OR/1
  [Cellj2i_17] -> Node13_OR/2
  Node13_OR/1 -> [Path_13]
  [Celli2j_17] -> Node14_OR/1
  [Cellj2i_18] -> Node14_OR/2
  Node14_OR/1 -> [Path_14]
  [AP] -> Node14_OR/3
  [Celli2j_18] -> [Path_15]
  [Celli2j_19] -> Node16_OR/1
  [Cellj2i_20] -> Node16_OR/2
  Node16_OR/1 -> [Path_16]
  [Celli2j_20] -> Node17_OR/1
  [Cellj2i_21] -> Node17_OR/2
  Node17_OR/1 -> [Path_17]
  [Celli2j_21] -> [Path_18]
  [Celli2j_15] -> Node19_OR/1
  [Celli2j_22] -> Node19_OR/2
  [Cellj2i_23] -> Node19_OR/3
  Node19_OR/1 -> [Path_19]
  [Celli2j_23] -> Node20_OR/1
  [Cellj2i_24] -> Node20_OR/2
  Node20_OR/1 -> [Path_20]
  [Celli2j_24] -> Node21_OR/1
  [Cellj2i_25] -> Node21_OR/2
  Node21_OR/1 -> [Path_21]
  [Celli2j_25] -> Node22_OR/1
  [Cellj2i_26] -> Node22_OR/2
  [Cellj2i_29] -> Node22_OR/3
  Node22_OR/1 -> [Path_22]
  [Celli2j_26] -> Node23_OR/1
  [Cellj2i_27] -> Node23_OR/2
  Node23_OR/1 -> [Path_23]
  [Celli2j_27] -> Node24_OR/1
  [Cellj2i_28] -> Node24_OR/2
  Node24_OR/1 -> [Path_24]
  [Celli2j_28] -> Node25_OR/1
  [Cellj2i_32] -> Node25_OR/2
  [Cellj2i_35] -> Node25_OR/3
  Node25_OR/1 -> [Path_25]
  [Celli2j_29] -> Node26_OR/1
  [Cellj2i_30] -> Node26_OR/2
  [Cellj2i_44] -> Node26_OR/3
  Node26_OR/1 -> [Path_26]
  [Celli2j_30] -> Node27_OR/1
  [Cellj2i_31] -> Node27_OR/2
  Node27_OR/1 -> [Path_27]
  [Celli2j_31] -> Node28_OR/1
  [Cellj2i_33] -> Node28_OR/2
  [Cellj2i_42] -> Node28_OR/3
  Node28_OR/1 -> [Path_28]
  [Celli2j_32] -> Node29_OR/1
  [Cellj2i_34] -> Node29_OR/2
  [Cellj2i_37] -> Node29_OR/3
  [Cellj2i_53] -> Node29_OR/4
  Node29_OR/1 -> [Path_29]
  [VP] -> Node29_OR/5
  [Celli2j_33] -> Node30_OR/1
  [Celli2j_34] -> Node30_OR/2
  [Cellj2i_39] -> Node30_OR/3
  [Cellj2i_51] -> Node30_OR/4
  Node30_OR/1 -> [Path_30]
  [Celli2j_37] -> Node31_OR/1
  [Cellj2i_38] -> Node31_OR/2
  [Cellj2i_46] -> Node31_OR/3
  Node31_OR/1 -> [Path_31]
  [Celli2j_38] -> Node32_OR/1
  [Cellj2i_45] -> Node32_OR/2
  Node32_OR/1 -> [Path_32]
  [Celli2j_35] -> Node33_OR/1
  [Cellj2i_36] -> Node33_OR/2
  [Cellj2i_47] -> Node33_OR/3
  Node33_OR/1 -> [Path_33]
  [Celli2j_36] -> Node34_OR/1
  [Cellj2i_48] -> Node34_OR/2
  Node34_OR/1 -> [Path_34]
  [Celli2j_40] -> Node35_OR/1
  [Cellj2i_41] -> Node35_OR/2
  [Celli2j_45] -> Node35_OR/3
  Node35_OR/1 -> [Path_35]
  [Celli2j_41] -> [Path_36]
  [Celli2j_39] -> Node37_OR/1
  [Cellj2i_40] -> Node37_OR/2
  [Celli2j_44] -> Node37_OR/3
  [Celli2j_46] -> Node37_OR/4
  Node37_OR/1 -> [Path_37]
  [Celli2j_42] -> Node38_OR/1
  [Cellj2i_43] -> Node38_OR/2
  [Cellj2i_49] -> Node38_OR/3
  Node38_OR/1 -> [Path_38]
  [Celli2j_43] -> Node39_OR/1
  [Cellj2i_50] -> Node39_OR/2
  Node39_OR/1 -> [Path_39]
  [Celli2j_47] -> Node40_OR/1
  [Celli2j_53] -> Node40_OR/2
  [Cellj2i_54] -> Node40_OR/3
  Node40_OR/1 -> [Path_40]
  [Celli2j_48] -> Node41_OR/1
  [Celli2j_54] -> Node41_OR/2
  Node41_OR/1 -> [Path_41]
  [Celli2j_49] -> Node42_OR/1
  [Celli2j_51] -> Node42_OR/2
  [Cellj2i_52] -> Node42_OR/3
  Node42_OR/1 -> [Path_42]
  [Celli2j_50] -> Node43_OR/1
  [Celli2j_52] -> Node43_OR/2
  Node43_OR/1 -> [Path_43]
  Cfgin/1 -> Cfg/1
  Pace/1 -> Pacing/1
  Cfg/1 -> [Para_1]
  Cfg/2 -> [Para_2]
  Cfg/3 -> [Para_3]
  Cfg/4 -> [Para_4]
  Cfg/5 -> [Para_5]
  Cfg/6 -> [Para_6]
  Cfg/7 -> [Para_7]
  Cfg/8 -> [Para_8]
  Cfg/9 -> [Para_9]
  Cfg/10 -> [Para_10]
  Cfg/11 -> [Para_11]
  Cfg/12 -> [Para_12]
  Cfg/13 -> [Para_13]
  Cfg/14 -> [Para_14]
  Cfg/15 -> [Para_15]
  Cfg/16 -> [Para_16]
  Cfg/17 -> [Para_17]
  Cfg/18 -> [Para_18]
  Cfg/19 -> [Para_19]
  Cfg/20 -> [Para_20]
  Cfg/21 -> [Para_21]
  Cfg/22 -> [Para_22]
  Cfg/23 -> [Para_23]
  Cfg/24 -> [Para_24]
  Cfg/25 -> [Para_25]
  Cfg/26 -> [Para_26]
  Cfg/27 -> [Para_27]
  Cfg/28 -> [Para_28]
  Cfg/29 -> [Para_29]
  Cfg/30 -> [Para_30]
  Cfg/31 -> [Para_31]
  Cfg/32 -> [Para_32]
  Cfg/33 -> [Para_33]
  Cfg/34 -> [Para_34]
  Cfg/35 -> [Para_35]
  Cfg/36 -> [Para_36]
  Cfg/37 -> [Para_37]
  Cfg/38 -> [Para_38]
  Cfg/39 -> [Para_39]
  Cfg/40 -> [Para_40]
  Cfg/41 -> [Para_41]
  Cfg/42 -> [Para_42]
  Cfg/43 -> [Para_43]
  Cfg/44 -> [Pcfg_1]
  Cfg/45 -> [Pcfg_2]
  Cfg/46 -> [Pcfg_3]
  Cfg/47 -> [Pcfg_4]
  Cfg/48 -> [Pcfg_5]
  Cfg/49 -> [Pcfg_6]
  Cfg/50 -> [Pcfg_7]
  Cfg/51 -> [Pcfg_8]
  Cfg/52 -> [Pcfg_9]
  Cfg/53 -> [Pcfg_10]
  Cfg/54 -> [Pcfg_11]
  Cfg/55 -> [Pcfg_12]
  Cfg/56 -> [Pcfg_13]
  Cfg/57 -> [Pcfg_14]
  Cfg/58 -> [Pcfg_15]
  Cfg/59 -> [Pcfg_16]
  Cfg/60 -> [Pcfg_17]
  Cfg/61 -> [Pcfg_18]
  Cfg/62 -> [Pcfg_19]
  Cfg/63 -> [Pcfg_20]
  Cfg/64 -> [Pcfg_21]
  Cfg/65 -> [Pcfg_22]
  Cfg/66 -> [Pcfg_23]
  Cfg/67 -> [Pcfg_24]
  Cfg/68 -> [Pcfg_25]
  Cfg/69 -> [Pcfg_26]
  Cfg/70 -> [Pcfg_27]
  Cfg/71 -> [Pcfg_28]
  Cfg/72 -> [Pcfg_29]
  Cfg/73 -> [Pcfg_30]
  Cfg/74 -> [Pcfg_31]
  Cfg/75 -> [Pcfg_32]
  Cfg/76 -> [Pcfg_33]
  Cfg/77 -> [Pcfg_34]
  Cfg/78 -> [Pcfg_35]
  Cfg/79 -> [Pcfg_36]
  Cfg/80 -> [Pcfg_37]
  Cfg/81 -> [Pcfg_38]
  Cfg/82 -> [Pcfg_39]
  Cfg/83 -> [Pcfg_40]
  Cfg/84 -> [Pcfg_41]
  Cfg/85 -> [Pcfg_42]
  Cfg/86 -> [Pcfg_43]
  Cfg/87 -> [Pcfg_44]
  Cfg/88 -> [Pcfg_45]
  Cfg/89 -> [Pcfg_46]
  Cfg/90 -> [Pcfg_47]
  Cfg/91 -> [Pcfg_48]
  Cfg/92 -> [Pcfg_49]
  Cfg/93 -> [Pcfg_50]
  Cfg/94 -> [Pcfg_51]
  Cfg/95 -> [Pcfg_52]
  Cfg/96 -> [Pcfg_53]
  Cfg/97 -> [Pcfg_54]
  Cfg/98 -> [Leads]
  Pacing/1 -> [AP]
  Pacing/2 -> [VP]
  Cell_out/1 -> Cells_out/1
  EGM_out/1 -> EGMs_out/1
  Wave_out/1 -> Waves_out/1
  [Cell_1] -> Cell_out/1
  [Cell_2] -> Cell_out/2
  [Cell_3] -> Cell_out/3
  [Cell_4] -> Cell_out/4
  [Cell_5] -> Cell_out/5
  [Cell_6] -> Cell_out/6
  [Cell_7] -> Cell_out/7
  [Cell_8] -> Cell_out/8
  [Cell_9] -> Cell_out/9
  [Cell_10] -> Cell_out/10
  [Cell_11] -> Cell_out/11
  [Cell_12] -> Cell_out/12
  [Cell_13] -> Cell_out/13
  [Cell_14] -> Cell_out/14
  [Cell_15] -> Cell_out/15
  [Cell_16] -> Cell_out/16
  [Cell_17] -> Cell_out/17
  [Cell_18] -> Cell_out/18
  [Cell_19] -> Cell_out/19
  [Cell_20] -> Cell_out/20
  [Cell_21] -> Cell_out/21
  [Cell_22] -> Cell_out/22
  [Cell_23] -> Cell_out/23
  [Cell_24] -> Cell_out/24
  [Cell_25] -> Cell_out/25
  [Cell_26] -> Cell_out/26
  [Cell_27] -> Cell_out/27
  [Cell_28] -> Cell_out/28
  [Cell_29] -> Cell_out/29
  [Cell_30] -> Cell_out/30
  [Cell_31] -> Cell_out/31
  [Cell_32] -> Cell_out/32
  [Cell_33] -> Cell_out/33
  [Cell_34] -> Cell_out/34
  [Cell_35] -> Cell_out/35
  [Cell_36] -> Cell_out/36
  [Cell_37] -> Cell_out/37
  [Cell_38] -> Cell_out/38
  [Cell_39] -> Cell_out/39
  [Cell_40] -> Cell_out/40
  [Cell_41] -> Cell_out/41
  [Cell_42] -> Cell_out/42
  [Cell_43] -> Cell_out/43
  [EGM_1] -> EGM_out/1
  [EGM_2] -> EGM_out/2
  [EGM_3] -> EGM_out/3
  [EGM_4] -> EGM_out/4
  [EGM_5] -> EGM_out/5
  [EGM_6] -> EGM_out/6
  [EGM_7] -> EGM_out/7
  [EGM_8] -> EGM_out/8
  [EGM_9] -> EGM_out/9
  [EGM_10] -> EGM_out/10
  [EGM_11] -> EGM_out/11
  [EGM_12] -> EGM_out/12
  [EGM_13] -> EGM_out/13
  [EGM_14] -> EGM_out/14
  [EGM_15] -> EGM_out/15
  [EGM_16] -> EGM_out/16
  [EGM_17] -> EGM_out/17
  [EGM_18] -> EGM_out/18
  [EGM_19] -> EGM_out/19
  [EGM_20] -> EGM_out/20
  [EGM_21] -> EGM_out/21
  [EGM_22] -> EGM_out/22
  [EGM_23] -> EGM_out/23
  [EGM_24] -> EGM_out/24
  [EGM_25] -> EGM_out/25
  [EGM_26] -> EGM_out/26
  [EGM_27] -> EGM_out/27
  [EGM_28] -> EGM_out/28
  [EGM_29] -> EGM_out/29
  [EGM_30] -> EGM_out/30
  [EGM_31] -> EGM_out/31
  [EGM_32] -> EGM_out/32
  [EGM_33] -> EGM_out/33
  [EGM_34] -> EGM_out/34
  [EGM_35] -> EGM_out/35
  [EGM_36] -> EGM_out/36
  [EGM_37] -> EGM_out/37
  [EGM_38] -> EGM_out/38
  [EGM_39] -> EGM_out/39
  [EGM_40] -> EGM_out/40
  [EGM_41] -> EGM_out/41
  [EGM_42] -> EGM_out/42
  [EGM_43] -> EGM_out/43
  [EGM_44] -> EGM_out/44
  [EGM_45] -> EGM_out/45
  [EGM_46] -> EGM_out/46
  [EGM_47] -> EGM_out/47
  [EGM_48] -> EGM_out/48
  [EGM_49] -> EGM_out/49
  [EGM_50] -> EGM_out/50
  [EGM_51] -> EGM_out/51
  [EGM_52] -> EGM_out/52
  [EGM_53] -> EGM_out/53
  [EGM_54] -> EGM_out/54
  [wave_1] -> Wave_out/1
  [wave_2] -> Wave_out/2
  [wave_3] -> Wave_out/3
  [wave_4] -> Wave_out/4
  [wave_5] -> Wave_out/5
  [wave_6] -> Wave_out/6
  [wave_7] -> Wave_out/7
  [wave_8] -> Wave_out/8
  [wave_9] -> Wave_out/9
  [wave_10] -> Wave_out/10
  [wave_11] -> Wave_out/11
  [wave_12] -> Wave_out/12
  [wave_13] -> Wave_out/13
  [wave_14] -> Wave_out/14
  [wave_15] -> Wave_out/15
  [wave_16] -> Wave_out/16
  [wave_17] -> Wave_out/17
  [wave_18] -> Wave_out/18
  [wave_19] -> Wave_out/19
  [wave_20] -> Wave_out/20
  [wave_21] -> Wave_out/21
  [wave_22] -> Wave_out/22
  [wave_23] -> Wave_out/23
  [wave_24] -> Wave_out/24
  [wave_25] -> Wave_out/25
  [wave_26] -> Wave_out/26
  [wave_27] -> Wave_out/27
  [wave_28] -> Wave_out/28
  [wave_29] -> Wave_out/29
  [wave_30] -> Wave_out/30
  [wave_31] -> Wave_out/31
  [wave_32] -> Wave_out/32
  [wave_33] -> Wave_out/33
  [wave_34] -> Wave_out/34
  [wave_35] -> Wave_out/35
  [wave_36] -> Wave_out/36
  [wave_37] -> Wave_out/37
  [wave_38] -> Wave_out/38
  [wave_39] -> Wave_out/39
  [wave_40] -> Wave_out/40
  [wave_41] -> Wave_out/41
  [wave_42] -> Wave_out/42
  [wave_43] -> Wave_out/43
  [wave_44] -> Wave_out/44
  [wave_45] -> Wave_out/45
  [wave_46] -> Wave_out/46
  [wave_47] -> Wave_out/47
  [wave_48] -> Wave_out/48
  [wave_49] -> Wave_out/49
  [wave_50] -> Wave_out/50
  [wave_51] -> Wave_out/51
  [wave_52] -> Wave_out/52
  [wave_53] -> Wave_out/53
  [wave_54] -> Wave_out/54

== stateflow chart CLSfixed/cfgs ==
  settings: executeAtInitialization=1
  state Ini
  state wait
  Ini -> wait : [t>800]{pUpdate(Paras);}
  (default) -> Ini : {Sensing=Scfgf;[Monitor, Pre]=Precfg;...
      |  [Heart] =LoadInit;}
  data: Scfg function_output; Mcfg function_output; Preout function_output; Parasin function_input; Hcfg function_output; Heart output; Sensing output; Monitor output; t input; Paras input; Pre output
  function Scfg= Scfgf:
    | function Scfg= Scfgf
    | 
    | %% desired
    | xa=1;
    | xc=0.05;
    | xc1=0.1;
    | xd=1;
    | xe=0.1;
    | avd=100;
    | vad=100;
    | uni_a=1;
    | Sens_a=0.6;
    | Amp_ap=500;
    | uni_v=1;
    | Sens_v=2.8;
    | Amp_vp=500;
    | 
    | Scfg=[xa xc xc1 xd xe avd vad uni_a Sens_a Amp_ap uni_v Sens_v Amp_vp]';
    | 
    | end
  function [Mcfg,Preout]= Precfg:
    | function [Mcfg,Preout]= Precfg
    | 
    | LRI=1000;
    | AVI=170;
    | URI=500;
    | VRP=230;
    | PVARP=250;
    | Mcfg=[LRI AVI URI VRP PVARP];
    | Preout=[VRP PVARP];
    | 
    | end
  function pUpdate(Parasin):
    | %% Get the index of the parameter
    | function pUpdate(Parasin)
    | %#codegen
    | coder.extrinsic('evalin');
    | coder.extrinsic('assignin');
    | Nodein=zeros(1,14); % The total number of cell cfg ports
    | Nodein=evalin('base', 'pNode');
    | Pathin=zeros(1,7); % The total number of path cfg ports
    | Pathin=evalin('base', 'pPath');
    | for n=1:length(Nodein)
    |     m=Nodein(n);
    |     Heart(m)=Parasin(n);
    | end
    | 
    | for n=1:length(Pathin)
    |     m=Pathin(n);
    |     nn=n+length(Nodein);
    |     Heart(m)=Parasin(nn);
    | end
    | 
    | assignin('base', 'Params', Parasin);
    | 
    | end
  function Hcfg   = LoadInit:
    | function Hcfg   = LoadInit
    | %#codegen
    | coder.extrinsic('evalin');
    | Hcfg1=zeros(1,2191); % The total number of cfg ports
    | Hcfg1=evalin('base', 'cfgdata');
    | Hcfg=Hcfg1';
    | end

== matlab function CLSfixed/newparas ==
  data: newparas output
function newparas= auto

coder.extrinsic('evalin');
coder.extrinsic('assignin');
newparas=zeros(1,21); % The total number of cell cfg ports
newparas=evalin('base', 'pp');

end

== stateflow chart CLSfixed/savedata ==
  settings: executeAtInitialization=1
  state termi
  state difa
  state Ini
  difa -> termi [order 1] : [rate_ave_a0>=60]/{coder.extrinsic('assignin');diffa=rate_ave_a1-rate_ave_a0;assignin('base', 'diffa', diffa);}
  (default) -> Ini : {rate_ave_vp=0; diffa=0;smax=0;}
  Ini -> difa [order 1] : [t>=29998]{coder.extrinsic('assignin','mean');assignin('base', 'reqqn', reqqn);assignin('base', 'errn', errn);assignin('base', 'smax', smax);...
      | assignin('base', 'errs', errs);assignin('base', 'reqs', reqs);assignin('base', 'reqqs', reqqs);...
      | assignin('base', 'nas0', nas0);assignin('base', 'nap0', nap0);assignin('base', 'nvs0', nvs0);assignin('base', 'nvp0', nvp0);...
      | assignin('base', 'rate_as0', rate_as0);assignin('base', 'rate_ap0', rate_ap0);assignin('base', 'rate_vs0', rate_vs0);assignin('base', 'rate_vp0', rate_vp0);...
      | assignin('base', 'nas1', nas1);assignin('base', 'nap1', nap1);assignin('base', 'nvs1', nvs1);assignin('base', 'nvp1', nvp1);...
      | assignin('base', 'rate_as1', rate_as1);assignin('base', 'rate_ap1', rate_ap1);assignin('base', 'rate_vs1', rate_vs1);assignin('base', 'rate_vp1', rate_vp1);...
      | rate_ave_vp=mean(rate_vp1(2,1:nvp1));assignin('base', 'rate_ave_vp', rate_ave_vp);...
      | rate_ave_a1=0;rate_ave_a1=mean([rate_as1(2,1:nas1) ]);rate_ave_a0=0;rate_ave_a0=mean(rate_as0(2,1:nas0));}
  difa -> termi [order 2] : [rate_ave_a0<60]/{coder.extrinsic('assignin');diffa=rate_ave_a1-60;assignin('base', 'diffa', diffa);}
  Ini -> Ini [order 2] : [s>smax]/{smax=s;}
  data: t input; reqqn input; errn input; s input; reqs input; errs input; reqqs input; nas0 input; nap0 input; nvs0 input; nvp0 input; rate_as0 input; rate_ap0 input; rate_vs0 input; rate_vp0 input; nas1 input; nap1 input; nvs1 input; nvp1 input; rate_as1 input; rate_ap1 input; rate_vs1 input; rate_vp1 input; diffa output double; rate_ave_a1 local double; rate_ave_vp output double; rate_ave_a0 local double; smax local
